simulink model "RBSdev"  (R2024a)
settings: Solver=VariableStepAuto  StartTime=0.0  StopTime=10.0  RelTol=1e-3
undefined symbols (not defined in the file): I_charge_max, Id, Id_char, Imax, Ion, Iq, lambda, Ld, Lithium, Lq, p, Rs, Soc_max, Tmax, V_batt, Vdc_nom, Vs_max
libraries: mcbcontrolslib x4, spsBatteryLib x1, simulink x1, spsPermanentMagnetSynchronousMachineLib x1, spsSeriesRLCBranchLib x1, spsThreePhaseFaultLib x1, spsUniversalBridgeLib x1, spspowerguiLib x1
(part 1 of 2)
settings Model: Creator=hirah  LastModifiedBy=hirah

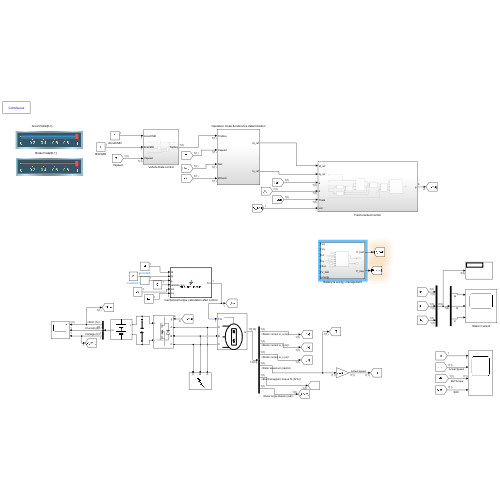
[thumbnail: Simulink's stored preview of the top-level diagram]
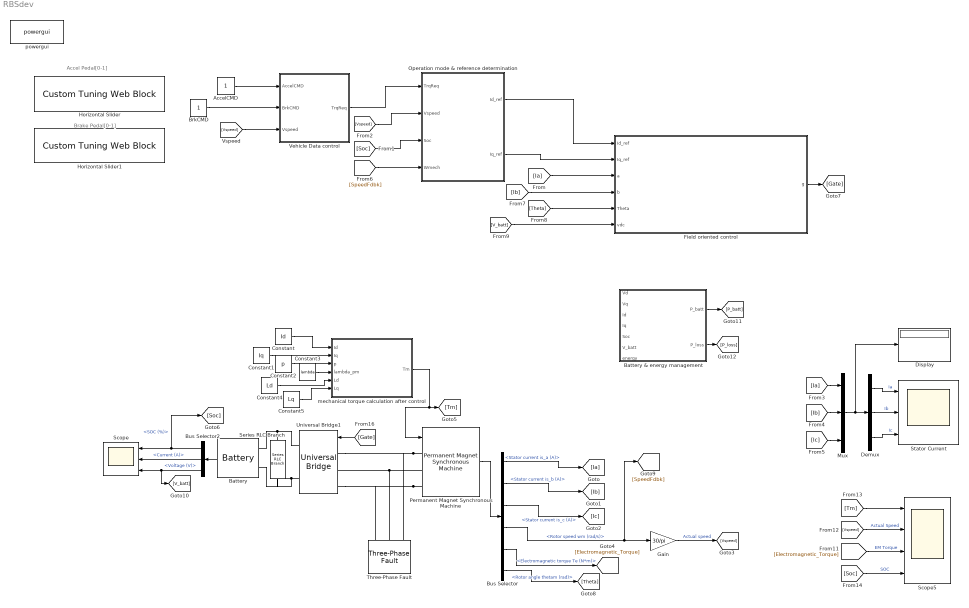
== system RBSdev ==
  note: Accel Pedal[0-1]
  note: Brake Pedal[0-1]
  AccelCMD : Constant
  Battery : spsBatteryLib/Battery  BatType=Lithium-Ion  ShowTempParam=off  ThermalPreset=no  ShowAgeParam=off  NomV=300  NomQ=100  SOC=80  Batt_Tr=30  PresetModel=off  MaxQ=84  MinV=215  FullV=330  Dis_rate=27.82608  R=0.006  Normal_OP=57.87524  expZone=[310 3.144344]  current=[1.5 3]  Units=Ampere-hour  Tci=20  NomT=20  T2=-30  MaxQ2=4.8  FullV2=7.1  Normal_OP2=5.655  expZone2="[6.58           1]"  Rca=0.6  ti=2000  Dp=0  Neq0=0  Tsim=1e6  Ta1=25  Qeol=5.4*0.9  Reol=0.013333*1.2  Char_age=[2.3478, 3]  Dis_age=[2.3478, 10]  N1=1500  N2=10500  N3=1000  N4=1400  Ta2=45  N5=950
  Battery & energy management : Subsystem
  BrkCMD : Constant
  Bus Selector : BusSelector  OutputSignals=Stator current is_a (A),Stator current is_b (A),Stator current is_c (A),Rotor speed wm (rad/s),Electromagnetic torque Te (N*m),Rotor angle thetam (rad)
  Bus Selector2 : BusSelector  OutputSignals=SOC (%),Current (A),Voltage (V)
  Constant : Constant  Value=Id
  Constant1 : Constant  Value=Iq
  Constant2 : Constant  Value=p
  Constant3 : Constant  Value=lambda
  Constant4 : Constant  Value=Ld
  Constant5 : Constant  Value=Lq
  Demux : Demux  Outputs=3
  Display : Display
  Field oriented control : Subsystem
  Gain : Gain  Gain=30/pi
  Horizontal Slider : CustomTuningWebBlock  LabelPosition=Hide  ShowInitialText=on  Configuration="{\"components\":[{\"name\":\"LinearScaleComponent\",\"settings\":{\"bounds\":{\"max\":1,\"min\":0,\"tickInterval\":\"auto\"},\"internalTickHeightScaleFactor\":0.5,\"labelColor\":[255,255,200],\"labelFont\":{\"font\":\"Arial\",\"fontSize\":12},\"labelOffset\":0.05,\"labelTransparency\":1,\"needleImage\":{\"size\":[596,842],\"src\":\"data:image\\/svg+xml;base64,PD94bWwgdmVyc2lvbj0iMS4wIiBlbmNvZGluZz0idXRmLTgiPz4NCjwhLS0gR2VuZXJhdG9yOiBBZG9iZSBJbGx1c3RyYXRvciAyNS4wLjAsIFNWRyBFeHBvcnQgUGx1Zy1JbiAuIFNWRyBWZXJzaW9uOiA2LjAwIEJ1aWxkIDApICAtLT4NCjxzdmcgdmVyc2lvbj0iMS4xIg0KCSBpZD0ic3ZnOCIgeG1sbnM6Y2M9Imh0dHA6Ly9jcmVhdGl2ZWNvbW1vbnMub3JnL25zIyIgeG1sbnM6ZGM9Imh0dHA6Ly9wdXJsLm9yZy9kYy9lbGVtZW50cy8xLjEvIiB4bWxuczppbmtzY2FwZT0iaHR0cDovL3d3dy5pbmtzY2FwZS5vcmcvbmFtZXNw ...(+2420 chars)\",\"srcOrientation\":\"Right\"},\"needleOffset\":[-0.8044596912521441,-0.0642123287671233],\"needleSize\":{\"height\":0.4337797619047619,\"width\":0.07668067226890757},\"position\":[0.2829861111111111,0.04398634453781513,0.9196428571428571,0.6088789682539683],\"referencePoint\":\"auto\",\"scaleColors\":[],\"scaleColorsSize\":0.2,\"scaleDirection\":\"LR\",\"showLabels\":1,\"showMinorTicks\":0,\"showSpanLine\":1,\"showTicks\":1,\"tickColor\":[252,252,197],\"tickTransparency\":1,\"valueBarColor\":[0,114,189],\"valueBarOffset\":-0.27,\"valueBarSize\":0.1,\"valueBarTransparency\":1}},{\"name\":\"BackgroundImageComponent\",\"settings\":{\"image\":{\"size\":[380,101],\"src\":\"data:image\\/svg+xml;base64,PHN2ZyB4bWxucz0iaHR0cDovL3d3dy53My5vcmcvMjAwMC9zdmciIHhtbG5zOnhsaW5rPSJodHRwOi8vd3d3LnczLm9yZy8xOTk5L3hsaW5rIiB2aWV3Qm94PSIwIDAgMzgwIDEwMSI+PGRlZnM+PHN0eWxlPi5jbHMtMXtmaWxsOiMwMDJiNDI7fS5jbHMtMntmaWxsOiM0MjcwODI7fS5jbHMtM3tmaWxsOnVybCgjcmFkaWFsLWdyYWRpZW50KTt9LmNscy00e2ZpbGw6I2M4YzhjODtzdHJva2U6IzAwMDt9PC9zdHlsZT48cmFkaWFsR3JhZGllbnQgaWQ9InJhZGlhbC1ncmFkaWVudCIgY3g9IjE5MCIgY3k9IjUwLjUiIHI9IjI2OS4yMSIgZ3JhZGllbnRVbml0cz0idXNlclNwYWNlT25Vc2UiPjxzdG9wIG9mZnNldD0iMC4wMSIgc3RvcC1jb2xvcj0iIzNlNGY1OCIvPjxzdG9wIG9mZnNldD0iMC4wNiIgc3RvcC1jb2xvcj0iIzQ0NTc2MSIvPjxzdG9wIG9mZnNldD0iMC4xNSIgc3RvcC1jb2xvcj0iIzU1NmE3NiIvPjxzdG9wIG9mZnNldD0iMC4yNSIgc3RvcC1jb2xvcj0iIzZkODg5NSIvPjxzdG9wIG9mZnNldD0iMC4zOCIgc3RvcC1jb2xvcj0iIzhmYjJjMyIvPjxzdG9wIG9mZnNldD0iMC41MiIgc3RvcC1jb2xvcj0iI2I2ZTRmYSIvPjxzdG9wIG9mZnNldD0iMSIgc3RvcC1jb2xvcj0iIzE1NDY1NyIvPjwvcmFkaWFsR3JhZGllbnQ+PC9kZWZzPjxnIGlkPSJmcmFtZSI+PGcgaWQ9IkxheWVyXzIiIGRhdGEtbmFtZT0iTGF5ZXIgMiI+PGcgaWQ9IkxheWVyXzEtMiIgZGF0YS1uYW1lPSJMYXllciAxLTIiPjxyZWN0IGlkPSJyZWN0MTAzNiIgY2xhc3M9ImNscy0xIiB4PSIxMSIgeT0iMTEiIHdpZHRoPSIzNTgiIGhlaWdodD0iNzkiLz48cGF0aCBpZD0icGF0aDEwMzgiIGNsYXNzPSJjbHMtMiIgZD0iTTgsOFY5M0gzNzJWOFpNMzY5LDkwSDExVjExSDM2OVoiLz48cGF0aCBpZD0icGF0aDEwNDAiIGNsYXNzPSJjbHMtMyIgZD0iTTAsMFYxMDFIMzgwVjBaTTM3Miw5M0g4VjhIMzcyWiIvPjwvZz48L2c+PC9nPjxnIGlkPSJ0cmFjayI+PHBhdGggaWQ9InJlY3QxNjExIiBjbGFzcz0iY2xzLTQiIGQ9Ik0zMy4zNywyNi41OUgzNDYuNjNjNCwwLDcuMjUsMi42LDcuMjUsNS44MWgwYzAsMy4yMS0zLjI1LDUuODItNy4yNSw1LjgySDMzLjM3Yy00LDAtNy4yNS0yLjYxLTcuMjUtNS44MmgwQzI2LjEyLDI5LjE5LDI5LjM3LDI2LjU5LDMzLjM3LDI2LjU5WiIvPjwvZz48L3N2Zz4=\",\"srcOrientation\":\"horizontal\"},\"position\":[0,0,1,1],\"scaleMode\":\"0\"}},{\"name\":\"ForegroundImageComponent\",\"settings\":{\"image\":{\"size\":[0,0],\"src\":\"default\",\"srcOrientation\":[]},\"isForeground\":1,\"position\":[0,0,1,1],\"scaleMode\":\"0\"}}],\"settings\":{\"BindingType\":\"param\",\"aspectRatio\":3.7777777777777777,\"backgroundColor\":[0,0,0,\"1\"],\"backgroundOffset\":0,\"backgroundOpacity\":1,\"fixedAspectRatio\":\"on\",\"foregroundColor\":[252,252,196],\"orientation\":\"horizontal\",\"showBackgroundColor\":false,\"value\":0,\"version\":\"R2023a\"},\"type\":\"LinearGauge\"}"
  Horizontal Slider1 : CustomTuningWebBlock  LabelPosition=Hide  ShowInitialText=on  Configuration="{\"components\":[{\"name\":\"LinearScaleComponent\",\"settings\":{\"bounds\":{\"max\":1,\"min\":0,\"tickInterval\":\"auto\"},\"internalTickHeightScaleFactor\":0.5,\"labelColor\":[255,255,200],\"labelFont\":{\"font\":\"Arial\",\"fontSize\":12},\"labelOffset\":0.05,\"labelTransparency\":1,\"needleImage\":{\"size\":[596,842],\"src\":\"data:image\\/svg+xml;base64,PD94bWwgdmVyc2lvbj0iMS4wIiBlbmNvZGluZz0idXRmLTgiPz4NCjwhLS0gR2VuZXJhdG9yOiBBZG9iZSBJbGx1c3RyYXRvciAyNS4wLjAsIFNWRyBFeHBvcnQgUGx1Zy1JbiAuIFNWRyBWZXJzaW9uOiA2LjAwIEJ1aWxkIDApICAtLT4NCjxzdmcgdmVyc2lvbj0iMS4xIg0KCSBpZD0ic3ZnOCIgeG1sbnM6Y2M9Imh0dHA6Ly9jcmVhdGl2ZWNvbW1vbnMub3JnL25zIyIgeG1sbnM6ZGM9Imh0dHA6Ly9wdXJsLm9yZy9kYy9lbGVtZW50cy8xLjEvIiB4bWxuczppbmtzY2FwZT0iaHR0cDovL3d3dy5pbmtzY2FwZS5vcmcvbmFtZXNw ...(+2420 chars)\",\"srcOrientation\":\"Right\"},\"needleOffset\":[-0.8044596912521441,-0.0642123287671233],\"needleSize\":{\"height\":0.4337797619047619,\"width\":0.07668067226890757},\"position\":[0.2829861111111111,0.04398634453781513,0.9196428571428571,0.6088789682539683],\"referencePoint\":\"auto\",\"scaleColors\":[],\"scaleColorsSize\":0.2,\"scaleDirection\":\"LR\",\"showLabels\":1,\"showMinorTicks\":0,\"showSpanLine\":1,\"showTicks\":1,\"tickColor\":[252,252,197],\"tickTransparency\":1,\"valueBarColor\":[0,114,189],\"valueBarOffset\":-0.27,\"valueBarSize\":0.1,\"valueBarTransparency\":1}},{\"name\":\"BackgroundImageComponent\",\"settings\":{\"image\":{\"size\":[380,101],\"src\":\"data:image\\/svg+xml;base64,PHN2ZyB4bWxucz0iaHR0cDovL3d3dy53My5vcmcvMjAwMC9zdmciIHhtbG5zOnhsaW5rPSJodHRwOi8vd3d3LnczLm9yZy8xOTk5L3hsaW5rIiB2aWV3Qm94PSIwIDAgMzgwIDEwMSI+PGRlZnM+PHN0eWxlPi5jbHMtMXtmaWxsOiMwMDJiNDI7fS5jbHMtMntmaWxsOiM0MjcwODI7fS5jbHMtM3tmaWxsOnVybCgjcmFkaWFsLWdyYWRpZW50KTt9LmNscy00e2ZpbGw6I2M4YzhjODtzdHJva2U6IzAwMDt9PC9zdHlsZT48cmFkaWFsR3JhZGllbnQgaWQ9InJhZGlhbC1ncmFkaWVudCIgY3g9IjE5MCIgY3k9IjUwLjUiIHI9IjI2OS4yMSIgZ3JhZGllbnRVbml0cz0idXNlclNwYWNlT25Vc2UiPjxzdG9wIG9mZnNldD0iMC4wMSIgc3RvcC1jb2xvcj0iIzNlNGY1OCIvPjxzdG9wIG9mZnNldD0iMC4wNiIgc3RvcC1jb2xvcj0iIzQ0NTc2MSIvPjxzdG9wIG9mZnNldD0iMC4xNSIgc3RvcC1jb2xvcj0iIzU1NmE3NiIvPjxzdG9wIG9mZnNldD0iMC4yNSIgc3RvcC1jb2xvcj0iIzZkODg5NSIvPjxzdG9wIG9mZnNldD0iMC4zOCIgc3RvcC1jb2xvcj0iIzhmYjJjMyIvPjxzdG9wIG9mZnNldD0iMC41MiIgc3RvcC1jb2xvcj0iI2I2ZTRmYSIvPjxzdG9wIG9mZnNldD0iMSIgc3RvcC1jb2xvcj0iIzE1NDY1NyIvPjwvcmFkaWFsR3JhZGllbnQ+PC9kZWZzPjxnIGlkPSJmcmFtZSI+PGcgaWQ9IkxheWVyXzIiIGRhdGEtbmFtZT0iTGF5ZXIgMiI+PGcgaWQ9IkxheWVyXzEtMiIgZGF0YS1uYW1lPSJMYXllciAxLTIiPjxyZWN0IGlkPSJyZWN0MTAzNiIgY2xhc3M9ImNscy0xIiB4PSIxMSIgeT0iMTEiIHdpZHRoPSIzNTgiIGhlaWdodD0iNzkiLz48cGF0aCBpZD0icGF0aDEwMzgiIGNsYXNzPSJjbHMtMiIgZD0iTTgsOFY5M0gzNzJWOFpNMzY5LDkwSDExVjExSDM2OVoiLz48cGF0aCBpZD0icGF0aDEwNDAiIGNsYXNzPSJjbHMtMyIgZD0iTTAsMFYxMDFIMzgwVjBaTTM3Miw5M0g4VjhIMzcyWiIvPjwvZz48L2c+PC9nPjxnIGlkPSJ0cmFjayI+PHBhdGggaWQ9InJlY3QxNjExIiBjbGFzcz0iY2xzLTQiIGQ9Ik0zMy4zNywyNi41OUgzNDYuNjNjNCwwLDcuMjUsMi42LDcuMjUsNS44MWgwYzAsMy4yMS0zLjI1LDUuODItNy4yNSw1LjgySDMzLjM3Yy00LDAtNy4yNS0yLjYxLTcuMjUtNS44MmgwQzI2LjEyLDI5LjE5LDI5LjM3LDI2LjU5LDMzLjM3LDI2LjU5WiIvPjwvZz48L3N2Zz4=\",\"srcOrientation\":\"horizontal\"},\"position\":[0,0,1,1],\"scaleMode\":\"0\"}},{\"name\":\"ForegroundImageComponent\",\"settings\":{\"image\":{\"size\":[0,0],\"src\":\"default\",\"srcOrientation\":[]},\"isForeground\":1,\"position\":[0,0,1,1],\"scaleMode\":\"0\"}}],\"settings\":{\"BindingType\":\"param\",\"aspectRatio\":3.7777777777777777,\"backgroundColor\":[0,0,0,\"1\"],\"backgroundOffset\":0,\"backgroundOpacity\":1,\"fixedAspectRatio\":\"on\",\"foregroundColor\":[252,252,196],\"orientation\":\"horizontal\",\"showBackgroundColor\":false,\"value\":0,\"version\":\"R2023a\"},\"type\":\"LinearGauge\"}"
  Mux : Mux  Inputs=3
  Operation mode & reference determination : Subsystem
  Permanent Magnet Synchronous Machine : spsPermanentMagnetSynchronousMachineLib/Permanent Magnet Synchronous Machine  NbPhases=3  FluxDistribution=Sinusoidal  RotorType=Round  MechanicalLoad=Torque Tm  PresetModel="07:  20 Nm 300 Vdc 2200 RPM - 33.9 Nm"  ShowDetailedParameters=on  MeasurementBus=off  Resistance=0.129  Inductance=0.0144e-3  dqInductances=[8.5e-3,8.5e-3]  La=0.00153  MachineConstant=Flux linkage established by magnets (V.s)  Flux=0.1821  VoltageCst=132.1171  TorqueCst=1.0926  Flat=120  Mechanical=[0.003334 0.000425 4 0]  PolePairs=4  InitialConditions=[0,0, 0,0]  InitialConditions5ph=[0 0 0 0 0 0]  RefAngle=90 degrees behind phase A axis (modified Park)  IterativeDiscreteModel=Trapezoidal non iterative  TsBlock=-1  TsPowergui=0
  Scope : Scope  NumInputPorts=3
  Scope5 : Scope  NumInputPorts=4
  Series RLC Branch : spsSeriesRLCBranchLib/Series RLC Branch  LConnTagsString=__new0  RConnTagsString=__new0  BranchType=C  Resistance=1  Inductance=1e-3  SetiL0=off  InitialCurrent=0  Capacitance=75e-3  Setx0=off  InitialVoltage=0  Measurements=None
  Stator Current : Scope  NumInputPorts=3
  Three-Phase Fault : spsThreePhaseFaultLib/Three-Phase Fault  InitialStates=0  FaultA=on  FaultB=on  FaultC=on  GroundFault=on  SwitchTimes="[1/60  5/60]"  External=off  SwitchStatus=NaN  FaultResistance=0.001  GroundResistance=0.01  SnubberResistance=1e6  SnubberCapacitance=inf  Measurements=None
  Universal Bridge1 : spsUniversalBridgeLib/Universal Bridge  Arms=3  SnubberResistance=1e5  SnubberCapacitance=inf  Device=MOSFET / Diodes  Ron=1e-3  Lon=0  ForwardVoltages="[  0  0  ]"  ForwardVoltage=0  GTOparameters=[ 10e-6 , 20e-6 ]  IGBTparameters=[ 1e-6 , 2e-6 ]  Measurements=None  Measurements_2=None  converterType=Rectifier
  Vehicle Data control : Subsystem
  mechanical torque calculation after control : MATLAB Function  TreatAsAtomicUnit=on
  powergui : spspowerguiLib/powergui  Priority=2  SimulationMode=Continuous  SampleTime=10e-6  frequency=60  Iterations=50  frequencyindice=0  Pbase=100e6  ErrMax=1e-4  UnitsV=kV  UnitsW=MW  buscounter=0  FunctionMessages=off  echomessages=off  EnableUseOfTLC=off  CurrentSourceSwitches=off  DisableSnubberDevices=off  DisableRonSwitches=off  DisableVfSwitches=off  DisplayEquations=off  AutomaticDiscreteSolvers=off  SolverType=Tustin  Interpol=off  ExternalGateDelay=off  methode=off  Ts=0  x0status=blocks  SPID=off  SwTol=0  HookPort=off  NonlinearTolerance=1e-4  nMaxIteration=100  ContinueOnMaxIteration=off  RestoreLinks=warning  ResistiveCurrentMeasurement=off  Frange=[0:2:500]  Ylog=off  Xlog=on  ShowGrid=off  save=off  variable=ZData  structure=N  ZoomFFT=off  StartTime=0.0  cycles=1  DisplayStyle=1  fundamental=60  FreqAxis=off  MaxFrequency=1000  frequencyindicesteady=1  RmsSteady=1  display=off
  wires:
  [Electromagnetic_Torque] -> Scope5/3  "EM Torque"
  Battery/1 -> Bus Selector2/1
  [Ib] -> Mux/2
  [Tm] -> Scope5/1
  Bus Selector2/3 -> [V_batt], Scope/3  "<Voltage (V)>"
  [Vspeed] -> Scope5/2  "Actual Speed"
  [Soc] -> Scope5/4  "SOC"
  Mux/1 -> Display/1, Demux/1
  Demux/1 -> Stator Current/1  "Ia"
  Bus Selector/2 -> [Ib]  "<Stator current is_b (A)>"
  [Gate] -> Universal Bridge1/1
  mechanical torque calculation after control/1(Tm) -> Permanent Magnet Synchronous Machine/1, [Tm]
  Bus Selector2/1 -> Scope/1, [Soc]  "<SOC (%)>"
  Permanent Magnet Synchronous Machine/1 -> Bus Selector/1
  Bus Selector/5 -> [Electromagnetic_Torque]  "<Electromagnetic torque Te (N*m)>"
  [Ic] -> Mux/3
  Bus Selector2/2 -> Scope/2  "<Current (A)>"
  Demux/2 -> Stator Current/2  "Ib"
  Gain/1 -> [Vspeed]  "Actual speed"
  Bus Selector/1 -> [Ia]  "<Stator current is_a (A)>"
  Demux/3 -> Stator Current/3  "Ic"
  Bus Selector/3 -> [Ic]  "<Stator current is_c (A)>"
  Bus Selector/4 -> [SpeedFdbk], Gain/1  "<Rotor speed wm (rad/s)>"
  [Ia] -> Mux/1
  [Vspeed] -> Vehicle Data control/3(Vspeed)
  BrkCMD/1 -> Vehicle Data control/2(BrkCMD)
  AccelCMD/1 -> Vehicle Data control/1(AccelCMD)
  Vehicle Data control/1(TrqReq) -> Operation mode & reference determination/1(TrqReq)
  Bus Selector/6 -> [Theta]  "<Rotor angle thetam (rad)>"
  [Soc] -> Operation mode & reference determination/3(Soc)
  [Vspeed] -> Operation mode & reference determination/2(Vspeed)
  [SpeedFdbk] -> Operation mode & reference determination/4(Wmech)
  Operation mode & reference determination/1(Id_ref) -> Field oriented control/1(Id_ref)
  Operation mode & reference determination/2(Iq_ref) -> Field oriented control/2(Iq_ref)
  [Ia] -> Field oriented control/3(a)
  [Ib] -> Field oriented control/4(b)
  [Theta] -> Field oriented control/5(Theta)
  [V_batt] -> Field oriented control/6(vdc)
  Field oriented control/1(g) -> [Gate]
  Constant/1 -> mechanical torque calculation after control/1(Id)
  Constant1/1 -> mechanical torque calculation after control/2(Iq)
  Constant2/1 -> mechanical torque calculation after control/3(p)
  Constant3/1 -> mechanical torque calculation after control/4(lambda_pm)
  Constant4/1 -> mechanical torque calculation after control/5(Ld)
  Constant5/1 -> mechanical torque calculation after control/6(Lq)
  Battery & energy management/1(P_batt) -> [P_batt]
  Battery & energy management/2(P_loss) -> [P_loss]
  connections:
  Universal Bridge1/RConn2 -- Series RLC Branch/RConn1 -- Battery/LConn2
  Three-Phase Fault/LConn2 -- Permanent Magnet Synchronous Machine/LConn2 -- Universal Bridge1/LConn2
  Battery/LConn1 -- Series RLC Branch/LConn1 -- Universal Bridge1/RConn1
  Permanent Magnet Synchronous Machine/LConn3 -- Universal Bridge1/LConn3 -- Three-Phase Fault/LConn3
  Permanent Magnet Synchronous Machine/LConn1 -- Universal Bridge1/LConn1 -- Three-Phase Fault/LConn1

== system RBSdev/Battery & energy management ==
  Vd : Inport
  Vq : Inport  Port=2
  Id : Inport  Port=3
  Iq : Inport  Port=4
  Soc : Inport  Port=5
  V_batt : Inport  Port=6
  energy : Inport  Port=7
  MATLAB Function : MATLAB Function  TreatAsAtomicUnit=on
  P_batt : Outport
  P_loss : Outport  Port=2
  wires:
  Vd/1 -> MATLAB Function/1(Vd)
  Vq/1 -> MATLAB Function/2(Vq)
  Id/1 -> MATLAB Function/3(Id)
  Iq/1 -> MATLAB Function/4(Iq)
  Soc/1 -> MATLAB Function/5(SOC)
  V_batt/1 -> MATLAB Function/6(V_batt)
  energy/1 -> MATLAB Function/7(energy)
  MATLAB Function/1(P_batt) -> P_batt/1
  MATLAB Function/2(P_loss) -> P_loss/1

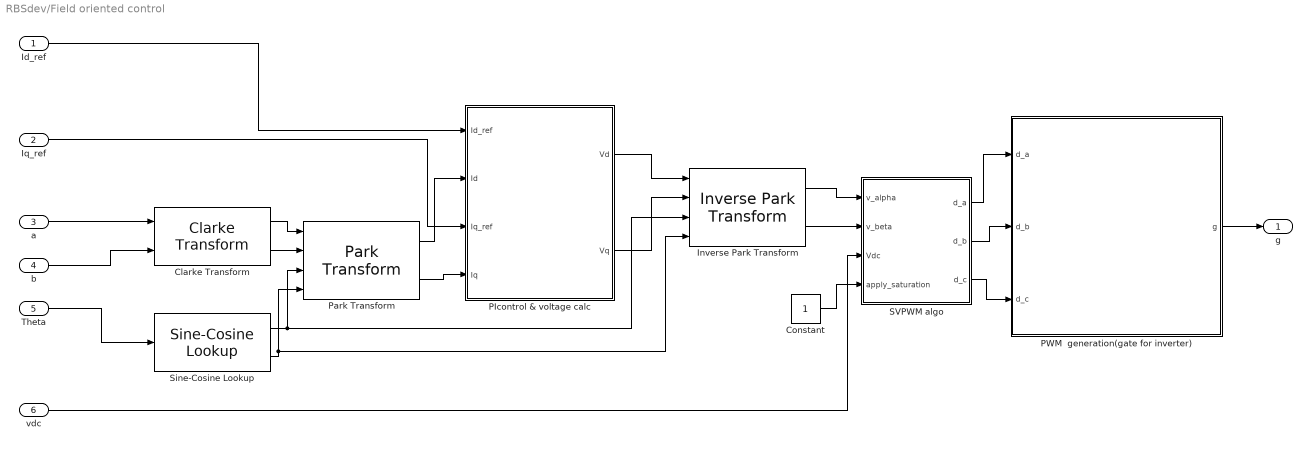
== system RBSdev/Field oriented control ==
  Id_ref : Inport
  Iq_ref : Inport  Port=2
  a : Inport  Port=3
  b : Inport  Port=4
  Theta : Inport  Port=5
  vdc : Inport  Port=6
  Clarke Transform : mcbcontrolslib/Clarke Transform  VariantControl=Variant2  PhaseInput=Two inputs  EnPowerInv=off
      settings: LibrarySourceBlock=mcbhdllib/Controls/Math Transforms/Clarke Transform
  Constant : Constant
  Inverse Park Transform : mcbcontrolslib/Inverse Park Transform  PhaseInput=Two inputs  AxisAlignment=D-axis  ThetaInput=Sine and Cosine electrical position  AngleInput=Per-unit  N_points=1024
      settings: LibrarySourceBlock=mcbhdllib/Controls/Math Transforms/Inverse Park Transform
  PIcontrol & voltage calc : MATLAB Function  TreatAsAtomicUnit=on
  PWM  generation(gate for inverter) : Subsystem
  Park Transform : mcbcontrolslib/Park Transform  PhaseInput=Two inputs  AxisAlignment=D-axis  ThetaInput=Sine and Cosine electrical position  AngleInput=Per-unit  N_points=1024
      settings: LibrarySourceBlock=mcbhdllib/Controls/Math Transforms/Park Transform
  SVPWM algo : MATLAB Function  TreatAsAtomicUnit=on
  Sine-Cosine Lookup : mcbcontrolslib/Sine-Cosine Lookup  AngleInput=Per-unit  N_points=1024  DatatypeInput=Inherit from input  Datatype=single
      settings: LibrarySourceBlock=mcblib/Controls/Math Transforms/Sine-Cosine Lookup
  g : Outport
  wires:
  b/1 -> Clarke Transform/2
  Clarke Transform/1 -> Park Transform/1
  a/1 -> Clarke Transform/1
  Sine-Cosine Lookup/2 -> Inverse Park Transform/4, Park Transform/4
  PIcontrol & voltage calc/1(Vd) -> Inverse Park Transform/1
  Clarke Transform/2 -> Park Transform/2
  Park Transform/1 -> PIcontrol & voltage calc/2(Id)
  Sine-Cosine Lookup/1 -> Inverse Park Transform/3, Park Transform/3
  PIcontrol & voltage calc/2(Vq) -> Inverse Park Transform/2
  Id_ref/1 -> PIcontrol & voltage calc/1(Id_ref)
  Park Transform/2 -> PIcontrol & voltage calc/4(Iq)
  Theta/1 -> Sine-Cosine Lookup/1
  Iq_ref/1 -> PIcontrol & voltage calc/3(Iq_ref)
  Inverse Park Transform/1 -> SVPWM algo/1(v_alpha)
  Inverse Park Transform/2 -> SVPWM algo/2(v_beta)
  vdc/1 -> SVPWM algo/3(Vdc)
  Constant/1 -> SVPWM algo/4(apply_saturation)
  SVPWM algo/1(d_a) -> PWM  generation(gate for inverter)/1(d_a)
  SVPWM algo/2(d_b) -> PWM  generation(gate for inverter)/2(d_b)
  SVPWM algo/3(d_c) -> PWM  generation(gate for inverter)/3(d_c)
  PWM  generation(gate for inverter)/1(g) -> g/1

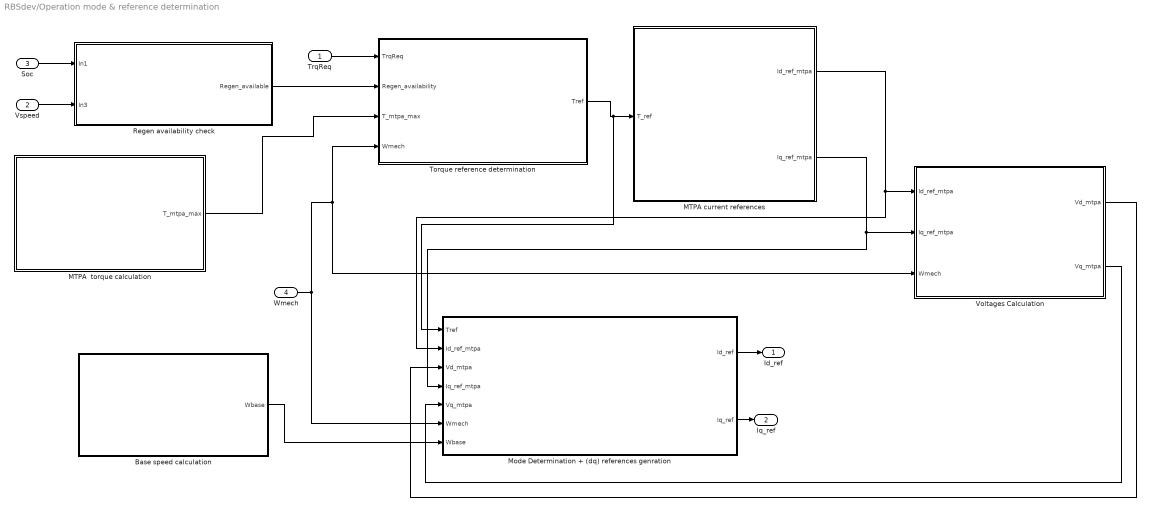
== system RBSdev/Operation mode & reference determination ==
  TrqReq : Inport
  Vspeed : Inport  Port=2
  Soc : Inport  Port=3
  Wmech : Inport  Port=4
  Base speed calculation : Subsystem
  MTPA  torque calculation : Subsystem
  MTPA current references : Subsystem
  Mode Determination + (dq) references genration : Subsystem
  Regen availability check : Subsystem
  Torque reference determination : Subsystem
  Voltages Calculation : Subsystem
  Id_ref : Outport
  Iq_ref : Outport  Port=2
  wires:
  Soc/1 -> Regen availability check/1(In1)
  Vspeed/1 -> Regen availability check/2(In3)
  Wmech/1 -> Mode Determination + (dq) references genration/6(Wmech), Voltages Calculation/3(Wmech), Torque reference determination/4(Wmech)
  TrqReq/1 -> Torque reference determination/1(TrqReq)
  Regen availability check/1(Regen_available) -> Torque reference determination/2(Regen_availability)
  MTPA  torque calculation/1(T_mtpa_max) -> Torque reference determination/3(T_mtpa_max)
  Torque reference determination/1(Tref) -> Mode Determination + (dq) references genration/1(Tref), MTPA current references/1(T_ref)
  MTPA current references/1(Id_ref_mtpa) -> Mode Determination + (dq) references genration/2(Id_ref_mtpa), Voltages Calculation/1(Id_ref_mtpa)
  MTPA current references/2(Iq_ref_mtpa) -> Mode Determination + (dq) references genration/4(Iq_ref_mtpa), Voltages Calculation/2(Iq_ref_mtpa)
  Voltages Calculation/1(Vd_mtpa) -> Mode Determination + (dq) references genration/3(Vd_mtpa)
  Voltages Calculation/2(Vq_mtpa) -> Mode Determination + (dq) references genration/5(Vq_mtpa)
  Base speed calculation/1(Wbase) -> Mode Determination + (dq) references genration/7(Wbase)
  Mode Determination + (dq) references genration/1(Id_ref) -> Id_ref/1
  Mode Determination + (dq) references genration/2(Iq_ref) -> Iq_ref/1

== system RBSdev/Vehicle Data control ==
  AccelCMD : Inport
  BrkCMD : Inport  Port=2
  Vspeed : Inport  Port=3
  Acceleration Pedal Characteristic : Lookup_n-D  NumberOfTableDimensions=1  BreakpointsForDimension1=[0 0.03 0.04 0.3 0.4 0.5 0.6 0.7 0.8 0.9 1]  Table=[0 0.04 0.07 0.1 0.15 0.2 0.3 0.4 0.6 0.8 1]*Tmax  InternalRulePriority=Speed  RndMeth=Simplest
  Brake Pedal Characteristic : Lookup_n-D  NumberOfTableDimensions=1  BreakpointsForDimension1=[0 0.03 0.04 0.3 0.4 0.5 0.6 0.7 0.8 0.9 1]  Table=[0, 0, -0.06, -0.10, -0.18, -0.25, -0.38, -0.47, -0.55, -0.63, -0.78]*(Tmax)  InternalRulePriority=Speed  RndMeth=Simplest
  Constant2 : Constant  Value=0  SampleTime=-1
  Sum : Sum  Inputs=|++
  v>0 : Switch  Criteria=u2 > Threshold  Threshold=0.1  SaturateOnIntegerOverflow=off  InputSameDT=off
  TrqReq : Outport  VectorParamsAs1DForOutWhenUnconnected=off
  wires:
  v>0/1 -> Sum/2
  Constant2/1 -> v>0/3
  Vspeed/1 -> v>0/2
  BrkCMD/1 -> Brake Pedal Characteristic/1
  Sum/1 -> TrqReq/1
  Brake Pedal Characteristic/1 -> v>0/1
  Acceleration Pedal Characteristic/1 -> Sum/1
  AccelCMD/1 -> Acceleration Pedal Characteristic/1

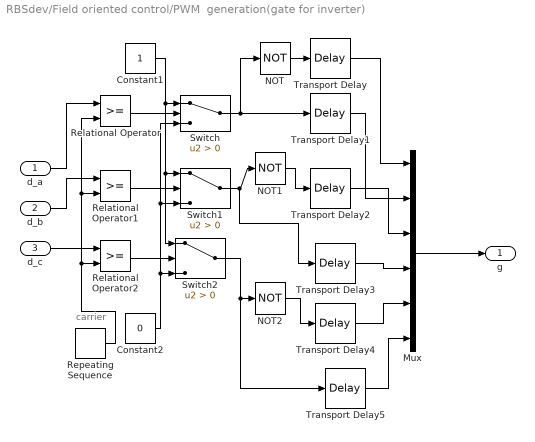
== system RBSdev/Field oriented control/PWM  generation(gate for inverter) ==
  note: carrier
  d_a : Inport
  d_b : Inport  Port=2
  d_c : Inport  Port=3
  Constant1 : Constant
  Constant2 : Constant  Value=0
  Mux : Mux  Inputs=6
  NOT : Logic  Operator=NOT  IconShape=distinctive  AllPortsSameDT=off  OutDataTypeStr=boolean
  NOT1 : Logic  Operator=NOT  IconShape=distinctive  AllPortsSameDT=off  OutDataTypeStr=boolean
  NOT2 : Logic  Operator=NOT  IconShape=distinctive  AllPortsSameDT=off  OutDataTypeStr=boolean
  Relational Operator : RelationalOperator  OutDataTypeStr=boolean  RndMeth=Simplest  InputSameDT=off
  Relational Operator1 : RelationalOperator  OutDataTypeStr=boolean  RndMeth=Simplest  InputSameDT=off
  Relational Operator2 : RelationalOperator  OutDataTypeStr=boolean  RndMeth=Simplest  InputSameDT=off
  Repeating Sequence : simulink/Sources/Repeating Sequence  rep_seq_t=[0, 0.5, 1]*1e-4  rep_seq_y=[0, 1, 0]
  Switch : Switch  Criteria=u2 > Threshold  SaturateOnIntegerOverflow=off  InputSameDT=off
  Switch1 : Switch  Criteria=u2 > Threshold  SaturateOnIntegerOverflow=off  InputSameDT=off
  Switch2 : Switch  Criteria=u2 > Threshold  SaturateOnIntegerOverflow=off  InputSameDT=off
  Transport Delay{,1..5} (6 alike) : TransportDelay  DelayTime=300e-9
  g : Outport
  wires:
  Repeating Sequence/1 -> Relational Operator2/2, Relational Operator1/2, Relational Operator/2
  NOT2/1 -> Transport Delay4/1
  Switch2/1 -> Transport Delay5/1, NOT2/1
  Transport Delay/1 -> Mux/1
  Constant1/1 -> Switch2/1, Switch1/1, Switch/1
  Mux/1 -> g/1
  NOT1/1 -> Transport Delay2/1
  Switch/1 -> Transport Delay1/1, NOT/1
  Constant2/1 -> Switch/3, Switch1/3, Switch2/3
  Switch1/1 -> Transport Delay3/1, NOT1/1
  Transport Delay2/1 -> Mux/3
  Transport Delay1/1 -> Mux/2
  Relational Operator/1 -> Switch/2
  NOT/1 -> Transport Delay/1
  d_c/1 -> Relational Operator2/1
  Transport Delay5/1 -> Mux/6
  Transport Delay3/1 -> Mux/4
  Transport Delay4/1 -> Mux/5
  Relational Operator1/1 -> Switch1/2
  Relational Operator2/1 -> Switch2/2
  d_a/1 -> Relational Operator/1
  d_b/1 -> Relational Operator1/1

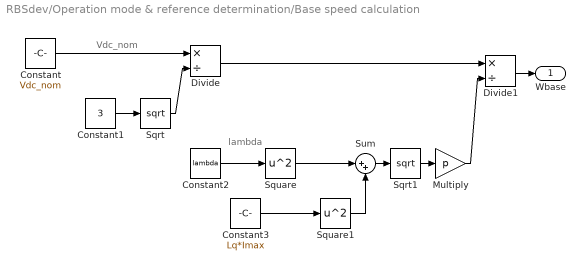
== system RBSdev/Operation mode & reference determination/Base speed calculation ==
  note: lambda
  note: Vdc_nom
  Constant : Constant  Value=Vdc_nom
  Constant1 : Constant  Value=3
  Constant2 : Constant  Value=lambda
  Constant3 : Constant  Value=Lq*Imax
  Divide : Product  Inputs=*/
  Divide1 : Product  Inputs=*/
  Multiply : Gain  Gain=p
  Sqrt : Sqrt
  Sqrt1 : Sqrt
  Square : Math  Operator=square
  Square1 : Math  Operator=square
  Sum : Sum  Inputs=|++
  Wbase : Outport
  wires:
  Sqrt1/1 -> Multiply/1
  Divide/1 -> Divide1/1
  Constant3/1 -> Square1/1
  Sum/1 -> Sqrt1/1
  Multiply/1 -> Divide1/2
  Square1/1 -> Sum/2
  Square/1 -> Sum/1
  Constant2/1 -> Square/1
  Constant1/1 -> Sqrt/1
  Sqrt/1 -> Divide/2
  Constant/1 -> Divide/1
  Divide1/1 -> Wbase/1

== system RBSdev/Operation mode & reference determination/MTPA  torque calculation ==
  Constant : Constant  Value=Imax
  Constant1 : Constant  Value=Ld
  Constant2 : Constant  Value=Lq
  Constant3 : Constant  Value=lambda
  MATLAB Function : MATLAB Function  TreatAsAtomicUnit=on
  T_mtpa_max : Outport
  wires:
  Constant1/1 -> MATLAB Function/2(Ld)
  Constant3/1 -> MATLAB Function/4(lambda_pm)
  Constant/1 -> MATLAB Function/1(I_max)
  MATLAB Function/1(T_mtpa_max) -> T_mtpa_max/1
  Constant2/1 -> MATLAB Function/3(Lq)

== system RBSdev/Operation mode & reference determination/MTPA current references ==
  T_ref : Inport
  Calculate MTPA reference currents : MATLAB Function  TreatAsAtomicUnit=on
  Constant : Constant  Value=Ld
  Constant1 : Constant  Value=Lq
  Constant2 : Constant  Value=lambda
  Id_ref_mtpa : Outport
  Iq_ref_mtpa : Outport  Port=2
  wires:
  Calculate MTPA reference currents/2(Iq_ref_mtpa) -> Iq_ref_mtpa/1
  Constant1/1 -> Calculate MTPA reference currents/3(Lq)
  Calculate MTPA reference currents/1(Id_ref_mtpa) -> Id_ref_mtpa/1
  Constant/1 -> Calculate MTPA reference currents/2(Ld)
  T_ref/1 -> Calculate MTPA reference currents/1(T_ref)
  Constant2/1 -> Calculate MTPA reference currents/4(lambda_pm)

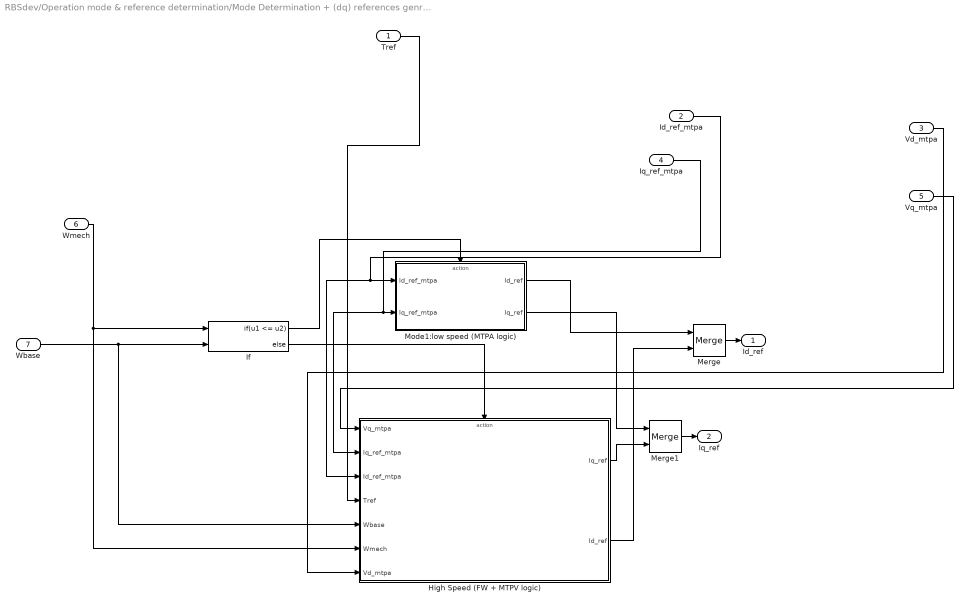
== system RBSdev/Operation mode & reference determination/Mode Determination + (dq) references genration ==
  Tref : Inport
  Id_ref_mtpa : Inport  Port=2
  Vd_mtpa : Inport  Port=3
  Iq_ref_mtpa : Inport  Port=4
  Vq_mtpa : Inport  Port=5
  Wmech : Inport  Port=6
  Wbase : Inport  Port=7
  High Speed (FW + MTPV logic) : Subsystem  TreatAsAtomicUnit=on
  If : If  NumInputs=2  IfExpression=u1 <= u2
  Merge : Merge
  Merge1 : Merge
  Mode1:low speed (MTPA logic) : Subsystem  TreatAsAtomicUnit=on
  Id_ref : Outport
  Iq_ref : Outport  Port=2
  wires:
  Wmech/1 -> High Speed (FW + MTPV logic)/6(Wmech), If/1
  If/2 -> High Speed (FW + MTPV logic)/Action
  Wbase/1 -> High Speed (FW + MTPV logic)/5(Wbase), If/2
  Mode1:low speed (MTPA logic)/1(Id_ref) -> Merge/1
  Mode1:low speed (MTPA logic)/2(Iq_ref) -> Merge1/1
  High Speed (FW + MTPV logic)/2(Id_ref) -> Merge/2
  High Speed (FW + MTPV logic)/1(Iq_ref) -> Merge1/2
  Iq_ref_mtpa/1 -> High Speed (FW + MTPV logic)/2(Iq_ref_mtpa), Mode1:low speed (MTPA logic)/2(Iq_ref_mtpa)
  If/1 -> Mode1:low speed (MTPA logic)/Action
  Id_ref_mtpa/1 -> High Speed (FW + MTPV logic)/3(Id_ref_mtpa), Mode1:low speed (MTPA logic)/1(Id_ref_mtpa)
  Vd_mtpa/1 -> High Speed (FW + MTPV logic)/7(Vd_mtpa)
  Vq_mtpa/1 -> High Speed (FW + MTPV logic)/1(Vq_mtpa)
  Tref/1 -> High Speed (FW + MTPV logic)/4(Tref)
  Merge1/1 -> Iq_ref/1
  Merge/1 -> Id_ref/1

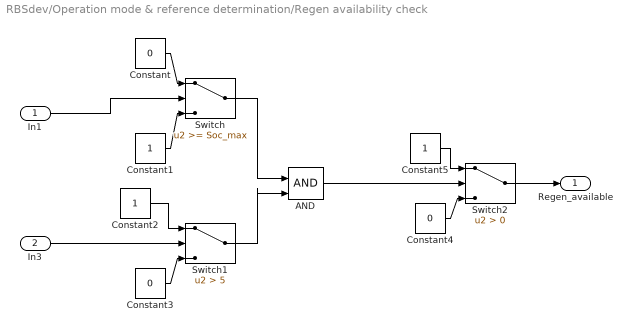
== system RBSdev/Operation mode & reference determination/Regen availability check ==
  In1 : Inport
  In3 : Inport  Port=2
  AND : Logic  IconShape=distinctive  AllPortsSameDT=off  OutDataTypeStr=boolean
  Constant : Constant  Value=0
  Constant1 : Constant
  Constant2 : Constant
  Constant3 : Constant  Value=0
  Constant4 : Constant  Value=0
  Constant5 : Constant
  Switch : Switch  Threshold=Soc_max  SaturateOnIntegerOverflow=off  InputSameDT=off
  Switch1 : Switch  Criteria=u2 > Threshold  Threshold=5  SaturateOnIntegerOverflow=off  InputSameDT=off
  Switch2 : Switch  Criteria=u2 > Threshold  SaturateOnIntegerOverflow=off  InputSameDT=off
  Regen_available : Outport
  wires:
  Constant1/1 -> Switch/3
  Constant4/1 -> Switch2/3
  Constant2/1 -> Switch1/1
  Constant3/1 -> Switch1/3
  Constant/1 -> Switch/1
  AND/1 -> Switch2/2
  Switch1/1 -> AND/2
  Switch/1 -> AND/1
  In3/1 -> Switch1/2
  Switch2/1 -> Regen_available/1
  In1/1 -> Switch/2
  Constant5/1 -> Switch2/1

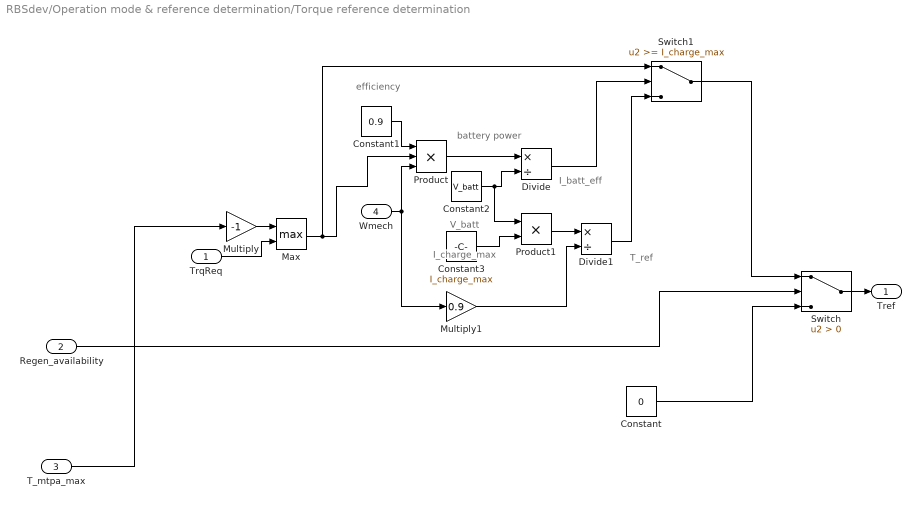
== system RBSdev/Operation mode & reference determination/Torque reference determination ==
  note: T_ref
  note: I_batt_eff
  note: V_batt
  note: I_charge_max
  note: battery power
  note: efficiency
  TrqReq : Inport
  Regen_availability : Inport  Port=2
  T_mtpa_max : Inport  Port=3
  Wmech : Inport  Port=4
  Constant : Constant  Value=0
  Constant1 : Constant  Value=0.9
  Constant2 : Constant  Value=V_batt
  Constant3 : Constant  Value=I_charge_max
  Divide : Product  Inputs=*/
  Divide1 : Product  Inputs=*/
  Max : MinMax  Function=max  Inputs=2
  Multiply : Gain  Gain=-1
  Multiply1 : Gain  Gain=0.9
  Product : Product  Inputs=3
  Product1 : Product
  Switch : Switch  Criteria=u2 > Threshold  SaturateOnIntegerOverflow=off  InputSameDT=off
  Switch1 : Switch  Threshold=I_charge_max  SaturateOnIntegerOverflow=off  InputSameDT=off
  Tref : Outport
  wires:
  Divide1/1 -> Switch1/3
  Multiply1/1 -> Divide1/2
  Max/1 -> Switch1/1, Product/2
  Wmech/1 -> Multiply1/1, Product/3
  Multiply/1 -> Max/1
  Constant2/1 -> Product1/1, Divide/2
  Product/1 -> Divide/1
  Constant1/1 -> Product/1
  Product1/1 -> Divide1/1
  Constant3/1 -> Product1/2
  Divide/1 -> Switch1/2
  Constant/1 -> Switch/3
  Switch1/1 -> Switch/1
  TrqReq/1 -> Max/2
  Switch/1 -> Tref/1
  T_mtpa_max/1 -> Multiply/1
  Regen_availability/1 -> Switch/2

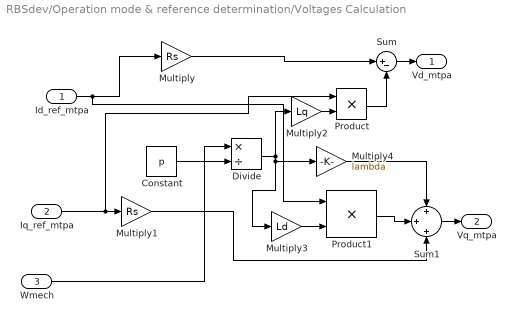
== system RBSdev/Operation mode & reference determination/Voltages Calculation ==
  Id_ref_mtpa : Inport
  Iq_ref_mtpa : Inport  Port=2
  Wmech : Inport  Port=3
  Constant : Constant  Value=p
  Divide : Product  Inputs=*/
  Multiply : Gain  Gain=Rs
  Multiply1 : Gain  Gain=Rs
  Multiply2 : Gain  Gain=Lq
  Multiply3 : Gain  Gain=Ld
  Multiply4 : Gain  Gain=lambda
  Product : Product
  Product1 : Product
  Sum : Sum  Inputs=|+-
  Sum1 : Sum  Inputs=+|+|+
  Vd_mtpa : Outport
  Vq_mtpa : Outport  Port=2
  wires:
  Iq_ref_mtpa/1 -> Product/1, Multiply1/1
  Id_ref_mtpa/1 -> Product1/1, Multiply/1
  Product/1 -> Sum/2
  Multiply/1 -> Sum/1
  Divide/1 -> Multiply4/1, Multiply3/1, Multiply2/1
  Constant/1 -> Divide/2
  Multiply2/1 -> Product/2
  Multiply4/1 -> Sum1/1
  Sum/1 -> Vd_mtpa/1
  Multiply3/1 -> Product1/2
  Wmech/1 -> Divide/1
  Product1/1 -> Sum1/2
  Multiply1/1 -> Sum1/3
  Sum1/1 -> Vq_mtpa/1

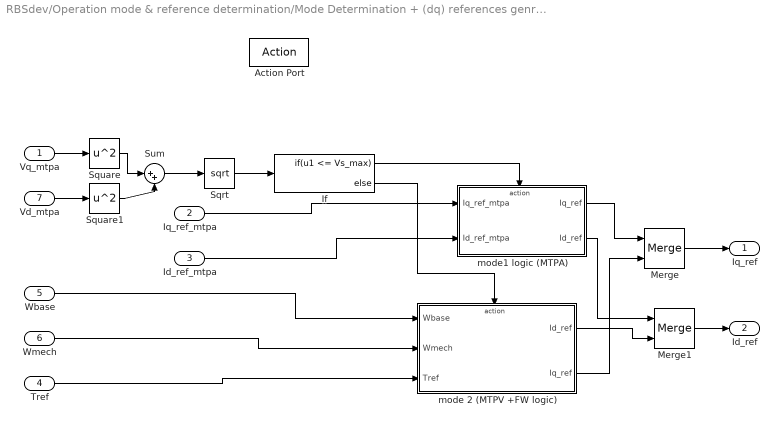
== system RBSdev/Operation mode & reference determination/Mode Determination + (dq) references genration/High Speed (FW + MTPV logic) ==
  Vq_mtpa : Inport
  Iq_ref_mtpa : Inport  Port=2
  Id_ref_mtpa : Inport  Port=3
  Tref : Inport  Port=4
  Wbase : Inport  Port=5
  Wmech : Inport  Port=6
  Vd_mtpa : Inport  Port=7
  Action Port : ActionPort  ActionPortLabel=else
  If : If  IfExpression=u1 <= Vs_max
  Merge : Merge
  Merge1 : Merge
  Sqrt : Sqrt
  Square : Math  Operator=square
  Square1 : Math  Operator=square
  Sum : Sum  Inputs=|++
  mode 2 (MTPV +FW logic) : Subsystem  TreatAsAtomicUnit=on
  mode1 logic (MTPA) : Subsystem  TreatAsAtomicUnit=on
  Iq_ref : Outport
  Id_ref : Outport  Port=2
  wires:
  Vq_mtpa/1 -> Square/1
  Vd_mtpa/1 -> Square1/1
  Square/1 -> Sum/1
  Square1/1 -> Sum/2
  Sum/1 -> Sqrt/1
  Sqrt/1 -> If/1
  If/1 -> mode1 logic (MTPA)/Action
  Iq_ref_mtpa/1 -> mode1 logic (MTPA)/1(Iq_ref_mtpa)
  Id_ref_mtpa/1 -> mode1 logic (MTPA)/2(Id_ref_mtpa)
  If/2 -> mode 2 (MTPV +FW logic)/Action
  Wbase/1 -> mode 2 (MTPV +FW logic)/1(Wbase)
  Wmech/1 -> mode 2 (MTPV +FW logic)/2(Wmech)
  Tref/1 -> mode 2 (MTPV +FW logic)/3(Tref)
  mode1 logic (MTPA)/1(Iq_ref) -> Merge/1
  mode 2 (MTPV +FW logic)/2(Iq_ref) -> Merge/2
  mode1 logic (MTPA)/2(Id_ref) -> Merge1/1
  mode 2 (MTPV +FW logic)/1(Id_ref) -> Merge1/2
  Merge/1 -> Iq_ref/1
  Merge1/1 -> Id_ref/1

== system RBSdev/Operation mode & reference determination/Mode Determination + (dq) references genration/Mode1:low speed (MTPA logic) ==
  Id_ref_mtpa : Inport
  Iq_ref_mtpa : Inport  Port=2
  Action Port : ActionPort  ActionPortLabel=if(u1 <= u2)
  mode1:low speed(MTPA refrences) : MATLAB Function  TreatAsAtomicUnit=on
  Id_ref : Outport
  Iq_ref : Outport  Port=2
  wires:
  Id_ref_mtpa/1 -> mode1:low speed(MTPA refrences)/1(Id_ref_mtpa)
  Iq_ref_mtpa/1 -> mode1:low speed(MTPA refrences)/2(Iq_ref_mtpa)
  mode1:low speed(MTPA refrences)/1(Iq_ref) -> Id_ref/1
  mode1:low speed(MTPA refrences)/2(Id_ref) -> Iq_ref/1

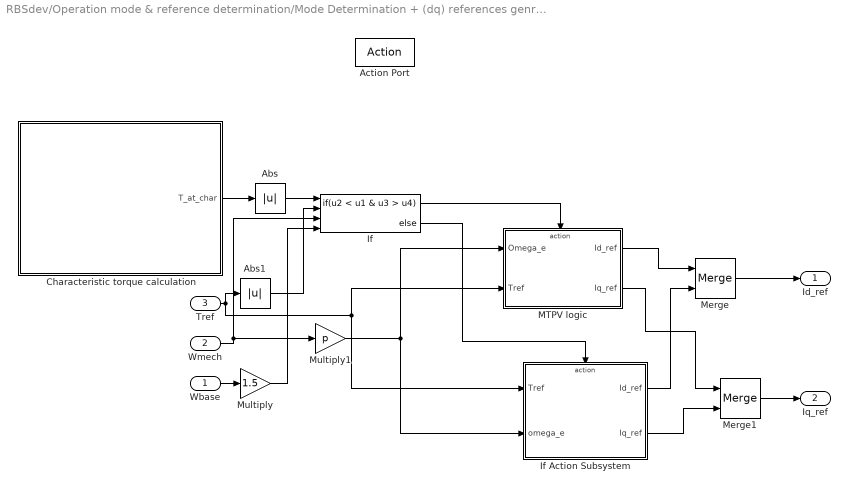
== system RBSdev/Operation mode & reference determination/Mode Determination + (dq) references genration/High Speed (FW + MTPV logic)/mode 2 (MTPV +FW logic) ==
  Wbase : Inport
  Wmech : Inport  Port=2
  Tref : Inport  Port=3
  Action Port : ActionPort  ActionPortLabel=else
  Abs : Abs  SaturateOnIntegerOverflow=off
  Abs1 : Abs  SaturateOnIntegerOverflow=off
  Characteristic torque calculation : Subsystem
  If : If  NumInputs=4  IfExpression=u2 < u1 & u3 > u4
  If Action Subsystem : Subsystem  TreatAsAtomicUnit=on
  MTPV logic : Subsystem  TreatAsAtomicUnit=on
  Merge : Merge
  Merge1 : Merge
  Multiply : Gain  Gain=1.5
  Multiply1 : Gain  Gain=p
  Id_ref : Outport
  Iq_ref : Outport  Port=2
  wires:
  Characteristic torque calculation/1(T_at_char) -> Abs/1
  Abs/1 -> If/1
  Wbase/1 -> Multiply/1
  Tref/1 -> Abs1/1, If Action Subsystem/1(Tref), MTPV logic/2(Tref)
  Abs1/1 -> If/2
  Wmech/1 -> Multiply1/1, If/3
  Multiply/1 -> If/4
  If/1 -> MTPV logic/Action
  Multiply1/1 -> If Action Subsystem/2(omega_e), MTPV logic/1(Omega_e)
  If/2 -> If Action Subsystem/Action
  If Action Subsystem/1(Id_ref) -> Merge/2
  MTPV logic/1(Id_ref) -> Merge/1
  If Action Subsystem/2(Iq_ref) -> Merge1/2
  MTPV logic/2(Iq_ref) -> Merge1/1
  Merge/1 -> Id_ref/1
  Merge1/1 -> Iq_ref/1

== system RBSdev/Operation mode & reference determination/Mode Determination + (dq) references genration/High Speed (FW + MTPV logic)/mode1 logic (MTPA) ==
  Iq_ref_mtpa : Inport
  Id_ref_mtpa : Inport  Port=2
  Action Port : ActionPort  ActionPortLabel=if(u1 <= Vs_max)
  Iq_ref : Outport
  Id_ref : Outport  Port=2
  wires:
  Iq_ref_mtpa/1 -> Iq_ref/1
  Id_ref_mtpa/1 -> Id_ref/1

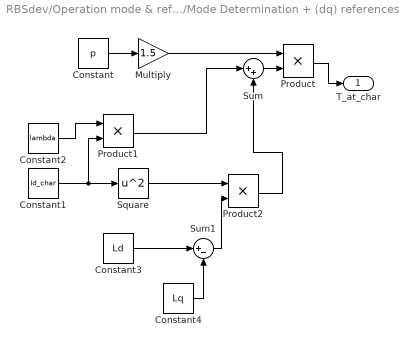
== system RBSdev/Operation mode & reference determination/Mode Determination + (dq) references genration/High Speed (FW + MTPV logic)/mode 2 (MTPV +FW logic)/Characteristic torque calculation ==
  Constant : Constant  Value=p
  Constant1 : Constant  Value=Id_char
  Constant2 : Constant  Value=lambda
  Constant3 : Constant  Value=Ld
  Constant4 : Constant  Value=Lq
  Multiply : Gain  Gain=1.5
  Product : Product
  Product1 : Product
  Product2 : Product
  Square : Math  Operator=square
  Sum : Sum  Inputs=|++
  Sum1 : Sum  Inputs=|+-
  T_at_char : Outport
  wires:
  Product1/1 -> Sum/1
  Product/1 -> T_at_char/1
  Sum1/1 -> Product2/2
  Constant3/1 -> Sum1/1
  Constant2/1 -> Product1/1
  Constant1/1 -> Square/1, Product1/2
  Sum/1 -> Product/2
  Product2/1 -> Sum/2
  Constant4/1 -> Sum1/2
  Square/1 -> Product2/1
  Multiply/1 -> Product/1
  Constant/1 -> Multiply/1

== system RBSdev/Operation mode & reference determination/Mode Determination + (dq) references genration/High Speed (FW + MTPV logic)/mode 2 (MTPV +FW logic)/If Action Subsystem ==
  Tref : Inport
  omega_e : Inport  Port=2
  Action Port : ActionPort  ActionPortLabel=else
  Constant : Constant  Value=Vs_max
  Constant1 : Constant  Value=Rs
  Constant2 : Constant  Value=Ld
  Constant3 : Constant  Value=Lq
  Constant4 : Constant  Value=lambda
  Constant5 : Constant  Value=Imax
  MATLAB Function : MATLAB Function  TreatAsAtomicUnit=on
  Id_ref : Outport
  Iq_ref : Outport  Port=2
  wires:
  Tref/1 -> MATLAB Function/1(T_ref)
  omega_e/1 -> MATLAB Function/3(omega_e)
  Constant/1 -> MATLAB Function/2(Vs_max)
  Constant1/1 -> MATLAB Function/4(Rs)
  Constant2/1 -> MATLAB Function/5(Ld)
  Constant3/1 -> MATLAB Function/6(Lq)
  Constant4/1 -> MATLAB Function/7(lambda_pm)
  Constant5/1 -> MATLAB Function/8(I_max)
  MATLAB Function/1(Id_ref) -> Id_ref/1
  MATLAB Function/2(Iq_ref) -> Iq_ref/1

== system RBSdev/Operation mode & reference determination/Mode Determination + (dq) references genration/High Speed (FW + MTPV logic)/mode 2 (MTPV +FW logic)/MTPV logic ==
  Omega_e : Inport
  Tref : Inport  Port=2
  Action Port : ActionPort  ActionPortLabel=if(u2 < u1 & u3 > u4)
  Constant : Constant  Value=Vs_max
  Constant1 : Constant  Value=Rs
  Constant2 : Constant  Value=Ld
  Constant3 : Constant  Value=Lq
  Constant4 : Constant  Value=lambda
  MATLAB Function : MATLAB Function  TreatAsAtomicUnit=on
  Id_ref : Outport
  Iq_ref : Outport  Port=2
  wires:
  Omega_e/1 -> MATLAB Function/3(omega_e)
  Tref/1 -> MATLAB Function/1(T_ref)
  Constant/1 -> MATLAB Function/2(Vs_max)
  Constant1/1 -> MATLAB Function/4(Rs)
  Constant2/1 -> MATLAB Function/5(Ld)
  Constant3/1 -> MATLAB Function/6(Lq)
  Constant4/1 -> MATLAB Function/7(lambda_pm)
  MATLAB Function/1(Id_ref) -> Id_ref/1
  MATLAB Function/2(Iq_ref) -> Iq_ref/1

== matlab function RBSdev/mechanical torque calculation after control ==
  data: Id input; Tm output; Iq input; p input; lambda_pm input; Ld input; Lq input
function Tm = calculate_torque(Id, Iq, p, lambda_pm, Ld, Lq)
% Calculate electromagnetic torque from dq currents
%
% Inputs:
%   Id       : d-axis current [A]
%   Iq       : q-axis current [A]
%   p        : pole pairs (3 for EQ CLA)
%   lambda_pm: PM flux linkage [Wb]
%   Ld       : d-axis inductance [H]
%   Lq       : q-axis inductance [H]
%
% Output:
%   Tm : Electromagnetic torque [Nm]

    % Magnetic torque + Reluctance torque
    Tm = 1.5 * p * (lambda_pm * Iq + (Ld - Lq) * Id * Iq);
    
    %  Breakdown:
    %  1.5 * p * lambda_pm * Iq  = magnetic torque  (from magnets)
    %  1.5 * p * (Ld-Lq) * Id*Iq = reluctance torque (from saliency)
    
end

== matlab function RBSdev/Battery & energy management/MATLAB Function ==
  data: Vd input; Vq input; Id input; Iq input; SOC input; V_batt input; energy input; P_batt output; P_loss output
% In your data.m or main script — just run section 6.10-6.12 directly:

%% Battery Update Function (standalone)
function [P_batt, P_loss] = ...
          update_battery(Vd, Vq, Id, Iq, SOC, V_batt, energy)

    % All parameters come from base workspace automatically
    % because this runs in the same script context
    
    global Rs V_batt_nom R_batt_int C_batt I_charge_max SOC_max dt

    %% 6.10
    P_motor  = 1.5 * (Vd*Id + Vq*Iq);
    P_switch = 0.02 * abs(P_motor);
    P_cond   = 1.5 * Rs * (Id^2 + Iq^2);
    P_loss   = P_switch + P_cond;
    P_batt   = P_motor - P_loss;
    I_batt   = P_batt / V_batt;

    if I_batt < I_charge_max
        I_batt = I_charge_max;
        P_batt = I_batt * V_batt;
    end

    V_batt = V_batt_nom - I_batt * R_batt_int;

    %% 6.11
    SOC = SOC + (-I_batt * dt / C_batt);
    SOC = min(max(SOC, 0), SOC_max);

    %% 6.12
    if P_batt < 0
        energy = energy + abs(P_batt) * dt;
    end
end

== matlab function RBSdev/Operation mode & reference determination/MTPA current references/Calculate MTPA reference currents ==
  data: T_ref input; Id_ref_mtpa output; Ld input; Lq input; lambda_pm input; Iq_ref_mtpa output
function [Id_ref_mtpa, Iq_ref_mtpa] = calculate_mtpa_currents(T_ref, Ld, Lq, lambda_pm)
    % Calculate MTPA current references for given torque
    % For negative torque (regen), Iq is negative
    T_norm = T_ref / 1.5;
    
    % MTPA trajectory: Id = f(Iq)
    % Solve: T_norm = λ_pm*Iq + (Ld-Lq)*Id*Iq for Id given T and Iq
    % Using MTPA condition
    
    if abs(T_ref) < 0.01
        Id_ref_mtpa = 0;
        Iq_ref_mtpa = 0;
        return;
    end
    
    % Analytical MTPA solution
    delta_L = Ld - Lq;  % Negative for IPMSM with Lq > Ld
    
    % For IPMSM, MTPA gives:
    % Id = -(λ_pm)/(2*delta_L) - sign(Iq)*sqrt((λ_pm/(2*delta_L))^2 + Iq^2)
    
    % Solve iteratively for Iq given T
    Iq_guess = T_norm / lambda_pm;  % Initial guess (ignoring reluctance)
    
    for iter = 1:50
        Id_guess = -(lambda_pm)/(2*delta_L) - sign(Iq_guess)*sqrt((lambda_pm/(2*delta_L))^2 + Iq_guess^2);
        T_calc = lambda_pm * Iq_guess + delta_L * Id_guess * Iq_guess;
        error = T_calc - T_norm;
        
        % Numerical derivative
        dIq = 0.1 * sign(Iq_guess);
        Id_plus = -(lambda_pm)/(2*delta_L) - sign(Iq_guess+dIq)*sqrt((lambda_pm/(2*delta_L))^2 + (Iq_guess+dIq)^2);
        T_plus = lambda_pm * (Iq_guess+dIq) + delta_L * Id_plus * (Iq_guess+dIq);
        dT_dIq = (T_plus - T_calc) / dIq;
        
        if abs(dT_dIq) > 1e-10
            Iq_guess = Iq_guess - error / dT_dIq;
        else
            break;
        end
        
        if abs(error) < 1e-6
            break;
        end
    end
    
    Id_ref_mtpa = -(lambda_pm)/(2*delta_L) - sign(Iq_guess)*sqrt((lambda_pm/(2*delta_L))^2 + Iq_guess^2);
    Iq_ref_mtpa = Iq_guess;
end

== matlab function RBSdev/Operation mode & reference determination/MTPA  torque calculation/MATLAB Function ==
  data: I_max input; T_mtpa_max output; Ld input; Lq input; lambda_pm input
function T_mtpa_max = calculate_mtpa_torque(I_max, Ld, Lq, lambda_pm)
    % Calculate maximum torque under MTPA with current limit
    % For IPMSM: T = 1.5*p*(λ_pm*Iq + (Ld-Lq)*Id*Iq)
    % MTPA condition: Id = -(λ_pm/(2*(Ld-Lq))) - sqrt((λ_pm/(2*(Ld-Lq)))^2 + Iq^2)
    
    Iq_range = linspace(0, I_max, 1000);
    T_range = zeros(size(Iq_range));
    Id_range = zeros(size(Iq_range));
    
    for j = 1:length(Iq_range)
        Iq_j = Iq_range(j);
        % MTPA Id for given Iq
        Id_j = -(lambda_pm/(2*(Ld-Lq))) - sqrt((lambda_pm/(2*(Ld-Lq)))^2 + Iq_j^2);
        % Check current limit
        if sqrt(Id_j^2 + Iq_j^2) <= I_max
            T_range(j) = 1.5 * (lambda_pm * Iq_j + (Ld - Lq) * Id_j * Iq_j);
            Id_range(j) = Id_j;
        end
    end
    
    [T_mtpa_max, idx] = max(T_range);
    %Id_opt = Id_range(idx);
    %Iq_opt = Iq_range(idx); %for current inspection and scope
end

== matlab function RBSdev/Operation mode & reference determination/Mode Determination + (dq) references genration/High Speed (FW + MTPV logic)/mode 2 (MTPV +FW logic)/MTPV logic/MATLAB Function ==
  data: T_ref input; Id_ref output; Vs_max input; omega_e input; Rs input; Ld input; Lq input; lambda_pm input; Iq_ref output
function [Id_ref, Iq_ref] = calculate_mptv_currents(T_ref, Vs_max, omega_e, Rs, Ld, Lq, lambda_pm)
    % Maximum Torque Per Voltage - voltage limited operation
    
    delta_L = Ld - Lq;
    T_norm = T_ref / 1.5;
    
    % MPTV occurs at the intersection of constant torque curve and voltage ellipse
    % with maximum Id (most negative) for that torque
    
    % Start from characteristic current
    Id_char = -lambda_pm / Lq;
    Id_guess = Id_char;
    Iq_guess = T_norm / (lambda_pm + delta_L * Id_char);
    
    for iter = 1:100
        % Voltage
        Vd = Rs*Id_guess - omega_e*Lq*Iq_guess;
        Vq = Rs*Iq_guess + omega_e*Ld*Id_guess + omega_e*lambda_pm;
        Vs = sqrt(Vd^2 + Vq^2);
        
        % Torque
        T_calc = lambda_pm * Iq_guess + delta_L * Id_guess * Iq_guess;
        
        err_V = Vs - Vs_max;
        err_T = T_calc - T_norm;
        
        % Adjust
        dId = 0.5;
        Vd_plus = Rs*(Id_guess+dId) - omega_e*Lq*Iq_guess;
        Vq_plus = Rs*Iq_guess + omega_e*Ld*(Id_guess+dId) + omega_e*lambda_pm;
        Vs_plus = sqrt(Vd_plus^2 + Vq_plus^2);
        dVs_dId = (Vs_plus - Vs) / dId;
        
        if abs(dVs_dId) > 1e-10
            Id_guess = Id_guess - err_V / dVs_dId;
        end
        
        if abs(lambda_pm + delta_L * Id_guess) > 1e-10
            Iq_guess = T_norm / (lambda_pm + delta_L * Id_guess);
        end
        
        if abs(err_V) < 0.1 && abs(err_T) < 0.01
            break;
        end
    end
    
    Id_ref = Id_guess;
    Iq_ref = Iq_guess;
end

== matlab function RBSdev/Operation mode & reference determination/Mode Determination + (dq) references genration/Mode1:low speed (MTPA logic)/mode1:low speed(MTPA refrences) ==
  data: Id_ref_mtpa input; Iq_ref output; Iq_ref_mtpa input; Id_ref output
function [Iq_ref,Id_ref] = get_mtpa_vals(Id_ref_mtpa,Iq_ref_mtpa)
    Is_ref = sqrt(Id_ref_mtpa^2 + Iq_ref_mtpa^2);
    if Is_ref > I_max
        Id_ref_mtpa = Id_ref_mtpa * I_max / Is_ref; %assure the references are always within the limits (limitation)
        Iq_ref_mtpa = Iq_ref_mtpa * I_max / Is_ref;
    end
    Id_ref = Id_ref_mtpa;
    Iq_ref = Iq_ref_mtpa;
end
